simulink model "ZT_VehCtrl_18B_CAN"  (R2018b)
settings: Solver=FixedStepAuto  StartTime=0.0  StopTime=inf  FixedStep=0.005  RelTol=1e-3
InitFcn:
  | mbd_mpc_consistency_checks(bdroot(gcs));
values from neighbouring files (symbols this model uses):
  BatoverTempTh = single(80)    [VCU_INIT.m]
  BRS_PwrValid = single(5)    [VCU_INIT.m]
  BRSEnSpdTh1 = single(10)    [VCU_INIT.m]
  BRSEnSpdTh2 = single(20)    [VCU_INIT.m]
  MCUTempAlarmTh = single (60)    [VCU_INIT.m]
  mps2kmh = single(3.6)    [VCU_INIT.m]
  MtrPwrFac = single(1/9550)    [VCU_INIT.m]
  MtrTempAlarmTh = single (50)    [VCU_INIT.m]
  Padle1Signal1_Th = [PadleSignal1_min,PadleSignal1_max]    [VCU_INIT.m]
  Padle1Signal2_Th = [PadleSignal2_min,PadleSignal2_max]    [VCU_INIT.m]
  PadleSignal1_max = 3.84    [VCU_INIT.m]
  PadleSignal1_min = 0.75    [VCU_INIT.m]
  PadleSignal2_max = 1.92    [VCU_INIT.m]
  PadleSignal2_min = 0.375    [VCU_INIT.m]
  PadleValid = 0.05    [VCU_INIT.m]
  PwrLimFactor = single(0.5)    [VCU_INIT.m]
  Ratio = single(1)    [VCU_INIT.m]
  rpm2mps = single(2*pi/60 * WhlRadius/Ratio)    [VCU_INIT.m]
  SOCLowTh = single(20)    [VCU_INIT.m]
  VehPwrBackwardMax = VehPwrMax * single(0.3)    [VCU_INIT.m]
  VehPwrMax = single(MtrPwrMax * 4)    [VCU_INIT.m]
  VehTrqBackwardMax = VehTrqMax * single(0.3)    [VCU_INIT.m]
  VehTrqMax = single(MtrTrqMax * Ratio *4)    [VCU_INIT.m]
  WhlRadius = single(1)    [VCU_INIT.m]
undefined symbols (not defined in the file or in its folder): Delay_Charge, Delay_Discharge, fifo_0_vect, fifo_1_vect, LQFP, pts1_fifo_0_vect, pts1_fifo_1_vect, pts2_fifo_0_vect, pts2_fifo_1_vect, pts3_fifo_0_vect, pts3_fifo_1_vect, pts4_fifo_0_vect, pts4_fifo_1_vect
libraries: mbd_mpc574x_ec_toolbox x157, canmsglib x74, simulink x38
(part 2 of 12)

== system ZT_VehCtrl_18B_CAN/Init ==
  CAN_init : Subsystem
  Data Store Read1 : DataStoreRead  DataStoreName=VCU_Mode
  Data Store Read3 : DataStoreRead  DataStoreName=Init_flg
  If1 : If  IfExpression=u1 == 2  ShowElse=off
  If2 : If  IfExpression=u1 == 0  ShowElse=off
  Init : Subsystem
  wires:
  Data Store Read3/1 -> If2/1
  If2/1 -> Init/Action
  Data Store Read1/1 -> If1/1
  If1/1 -> CAN_init/Action

== system ZT_VehCtrl_18B_CAN/Initialization & SPI timer1 ==
  note: 由于SPI0用了两个片选，SPI3只用了一个片选（没算EEPROM）。
      | 因此直接用方波就可以了。
      | 如果增加SPI控制，建议使用StateFlow构造激活函数。
      | 由于模版使用的0.01s的仿真步长，这里构造周期为0.02s,占空比为0.5的方波。
  note: SPI3
  note: SPI0
  CS1 LS : Subsystem
  CS2 CANB : Subsystem
  CS3 LS : Subsystem
  CS5 LS : Subsystem
  Chart : Stateflow chart  TreatAsAtomicUnit=on
  Chart1 : Stateflow chart  TreatAsAtomicUnit=on
  Chart2 : Stateflow chart  TreatAsAtomicUnit=on
  Compare To Constant : simulink/Logic and Bit Operations/Compare To Constant  relop===  const=9  OutDataTypeStr=boolean
  Compare To Constant1 : simulink/Logic and Bit Operations/Compare To Constant  relop===  const=9  OutDataTypeStr=boolean
  Constant : Constant
  Data Store Read : DataStoreRead  DataStoreName=VCU_Mode
  Data Store Read1 : DataStoreRead  DataStoreName=ResetFlg
  Data Store Read2 : DataStoreRead  DataStoreName=Init_flg_SPI
  Data Store Write : DataStoreWrite  DataStoreName=VCU_Mode
  Data Store Write2 : DataStoreWrite  DataStoreName=SPI0_CS
  Data Store Write3 : DataStoreWrite  DataStoreName=SPI3_CS
  Data Store Write4 : DataStoreWrite  DataStoreName=Init_flg_SPI
  Data Type Conversion{,1..3} (4 alike) : DataTypeConversion
  If : If  IfExpression=u1 == 1  ShowElse=off
  If1 : If  IfExpression=u1 == 1  ShowElse=off
  If2 : If  IfExpression=u1 == 2  ShowElse=off
  If3 : If  IfExpression=u1 == 2  ShowElse=off
  Logical Operator : Logic  AllPortsSameDT=off  OutDataTypeStr=boolean
  Pulse Generator : DiscretePulseGenerator  PulseType=Time based  Period=0.01  PulseWidth=50
  wires:
  If/1 -> CS2 CANB/Action
  Chart/1(Flg) -> Data Type Conversion3/1
  Data Store Read2/1 -> Chart/2(InitFlg)
  If1/1 -> CS1 LS/Action
  Chart2/1(Flg) -> If3/1, [SPI3_flg], If/1
  Data Store Read/1 -> Chart2/1(VcuMode), Chart1/1(VcuMode)
  If2/1 -> CS5 LS/Action
  [SPI0_flg] -> Compare To Constant/1
  [SPI3_flg] -> Compare To Constant1/1
  Compare To Constant/1 -> Logical Operator/1
  Compare To Constant1/1 -> Logical Operator/2
  Logical Operator/1 -> Data Type Conversion2/1
  If3/1 -> CS3 LS/Action
  Pulse Generator/1 -> Data Type Conversion/1
  Constant/1 -> Data Type Conversion1/1
  Data Type Conversion/1 -> Data Store Write2/1
  Data Type Conversion1/1 -> Data Store Write3/1
  Data Type Conversion2/1 -> Data Store Write4/1
  Data Type Conversion3/1 -> Data Store Write/1
  Chart1/1(Flg) -> If1/1, [SPI0_flg], If2/1
  Data Store Read1/1 -> Chart/1(ResetFlg)

== system ZT_VehCtrl_18B_CAN/Power Managment ==
  PowerMode : Inport
  Data Type Conversion : DataTypeConversion
  HS1 : mbd_mpc574x_ec_toolbox/GPIO Blocks/Digital_Output  Priority=1  gpio_pin=PTF6: [SIUL2_GPIO86 | General Purpose IO PF[6]]  gpio_drive_strength=Disabled
  HS4 : mbd_mpc574x_ec_toolbox/GPIO Blocks/Digital_Output  Priority=1  gpio_pin=PTA13: [SIUL2_GPIO13 | General Purpose IO PA[13]]  gpio_drive_strength=Disabled
  wires:
  PowerMode/1 -> Data Type Conversion/1
  Data Type Conversion/1 -> HS4/1, HS1/1

== system ZT_VehCtrl_18B_CAN/SPI_EEPROM ==
  Data Store Memory : DataStoreMemory  DataStoreName=A_write  ReadBeforeWriteMsg=warning  WriteAfterWriteMsg=warning  WriteAfterReadMsg=warning  ShowAdditionalParam=off  OutDataTypeStr=single
      settings: RTWStateStorageClass=ExportedGlobal
  Data Store Memory10 : DataStoreMemory  DataStoreName=A_read  ReadBeforeWriteMsg=warning  WriteAfterWriteMsg=warning  WriteAfterReadMsg=warning  ShowAdditionalParam=off  OutDataTypeStr=single
      settings: RTWStateStorageClass=ExportedGlobal
  Data Store Memory18 : DataStoreMemory  DataStoreName=SPI0_CTRL0  ReadBeforeWriteMsg=warning  WriteAfterWriteMsg=warning  WriteAfterReadMsg=warning  ShowAdditionalParam=off  OutDataTypeStr=uint8
      settings: RTWStateStorageClass=ExportedGlobal
  Data Store Read : DataStoreRead  DataStoreName=SPI0_CTRL0
  SPI_read : Subsystem  TreatAsAtomicUnit=on
  SPI_write : Subsystem  TreatAsAtomicUnit=on
  Switch Case : SwitchCase  CaseConditions={1,2}  ShowDefaultCase=off
  wires:
  Data Store Read/1 -> Switch Case/1
  Switch Case/2 -> SPI_write/Action
  Switch Case/1 -> SPI_read/Action

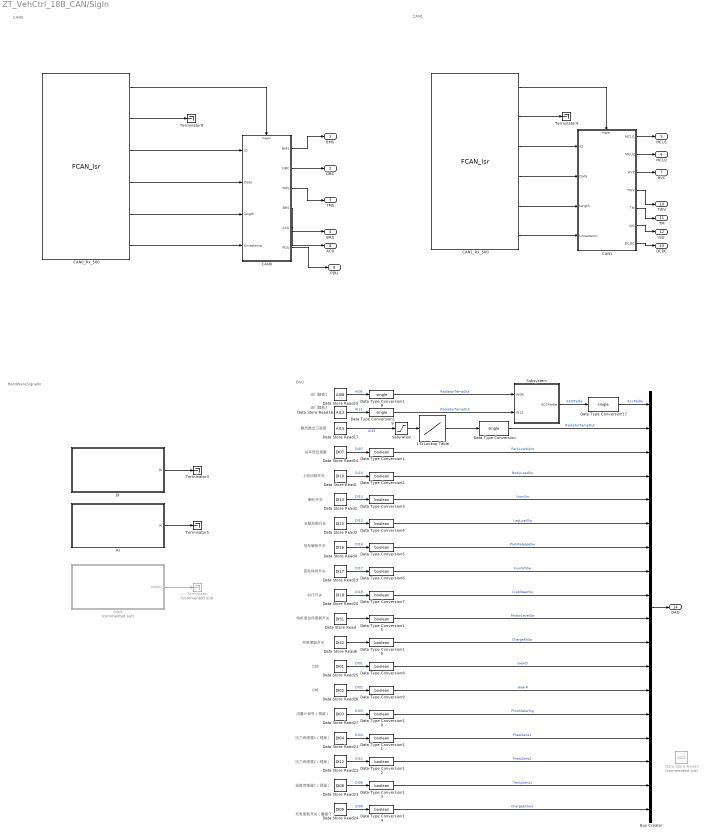
== system ZT_VehCtrl_18B_CAN/SigIn ==
  note: 充电使能开关（重复了）
  note: 温度传感器1（预留）
  note: 压力传感器2（预留）
  note: 压力传感器1（预留）
  note: 流量计信号（预留）
  note: R档
  note: D档
  note: 充电使能开关
  note: 电机液位传感器开关
  note: 斜行开关
  note: 四轮转向开关
  note: 驻车解除开关
  note: 支腿加载开关
  note: 喇叭开关
  note: 上装加载开关
  note: 驻车低压报警
  note: 散热器出口温度
  note: 油门踏板1
  note: DAQ
  note: CAN0
  note: HardWareSignalIn
  note: CAN1
  note: 油门踏板2
  1-D Lookup Table : Lookup_n-D  NumberOfTableDimensions=1  BreakpointsForDimension1=[0,5]  Table=[0,100]  InternalRulePriority=Speed  RndMeth=Simplest  InputSameDT=on
  AI : Subsystem
  Bus Creator : BusCreator  Inputs=18
  "CAN0 " : Subsystem  TreatAsAtomicUnit=on
      settings: RTWSystemCode=Nonreusable function
  CAN0_Rx_500 : mbd_mpc574x_ec_toolbox/Communication Blocks/CAN Blocks/FCAN_Isr  can_instance=0  can_event=Rx Complete
      settings: SourceProductName=NXP Model-Based Design Toolbox for MPC57xx MCUs
  CAN1 : Subsystem  TreatAsAtomicUnit=on
      settings: RTWSystemCode=Nonreusable function
  CAN1_Rx_500 : mbd_mpc574x_ec_toolbox/Communication Blocks/CAN Blocks/FCAN_Isr  can_instance=1  can_event=Rx Complete
      settings: SourceProductName=NXP Model-Based Design Toolbox for MPC57xx MCUs
  DI : Subsystem
  Data Store Read : DataStoreRead  DataStoreName=DI31
  Data Store Read1 : DataStoreRead  DataStoreName=DI10
  Data Store Read14 : DataStoreRead  DataStoreName=DI07
  Data Store Read15 : DataStoreRead  DataStoreName=AI08
  Data Store Read16 : DataStoreRead  DataStoreName=AI12
  Data Store Read17 : DataStoreRead  DataStoreName=AI15
  Data Store Read19 : DataStoreRead  DataStoreName=DI17
  Data Store Read2 : DataStoreRead  DataStoreName=DI13
  Data Store Read20 : DataStoreRead  DataStoreName=DI18
  Data Store Read21 : DataStoreRead  DataStoreName=DI04
  Data Store Read22 : DataStoreRead  DataStoreName=DI12
  Data Store Read23 : DataStoreRead  DataStoreName=DI08
  Data Store Read24 : DataStoreRead  DataStoreName=DI09
  Data Store Read25 : DataStoreRead  DataStoreName=DI01
  Data Store Read26 : DataStoreRead  DataStoreName=DI02
  Data Store Read27 : DataStoreRead  DataStoreName=DI03
  Data Store Read3 : DataStoreRead  DataStoreName=DI15
  Data Store Read4 : DataStoreRead  DataStoreName=DI16
  Data Store Read5 : DataStoreRead  Commented=on  DataStoreName=AI20
  Data Store Read6 : DataStoreRead  DataStoreName=DI32
  Data Type Conversion{,17..19} (4 alike) : DataTypeConversion  OutDataTypeStr=single
  Data Type Conversion{1..16} (16 alike) : DataTypeConversion  OutDataTypeStr=boolean
  PWM : Subsystem  Commented=on
  Saturation : Saturate
  Subsystem : Subsystem
  Terminator : Terminator  Commented=on
  Terminator{3..5,8} (4 alike) : Terminator
  BMS : Outport  VectorParamsAs1DForOutWhenUnconnected=on
  OBC : Outport  Port=2  VectorParamsAs1DForOutWhenUnconnected=on
  TMS : Outport  Port=3  VectorParamsAs1DForOutWhenUnconnected=on
  BRS : Outport  Port=4  VectorParamsAs1DForOutWhenUnconnected=on
  MCU1 : Outport  Port=5  VectorParamsAs1DForOutWhenUnconnected=on
  MCU2 : Outport  Port=6  VectorParamsAs1DForOutWhenUnconnected=on
  HVC : Outport  Port=7  VectorParamsAs1DForOutWhenUnconnected=on
  ACU : Outport  Port=8  VectorParamsAs1DForOutWhenUnconnected=on
  PDU : Outport  Port=9  VectorParamsAs1DForOutWhenUnconnected=on
  TWV : Outport  Port=10  VectorParamsAs1DForOutWhenUnconnected=on
  TM : Outport  Port=11  VectorParamsAs1DForOutWhenUnconnected=on
  ISG : Outport  Port=12  VectorParamsAs1DForOutWhenUnconnected=on
  DCDC : Outport  Port=13  VectorParamsAs1DForOutWhenUnconnected=on
  "DAQ " : Outport  Port=14
  wires:
  CAN1_Rx_500/2 -> Terminator4/1
  CAN1_Rx_500/6 -> CAN1/4(timestamp)
  CAN1_Rx_500/4 -> CAN1/2(Data)
  CAN1_Rx_500/3 -> CAN1/1(ID)
  CAN1_Rx_500/5 -> CAN1/3(length)
  CAN0_Rx_500/5 -> "CAN0 "/3(length)
  CAN0_Rx_500/3 -> "CAN0 "/1(ID)
  CAN0_Rx_500/4 -> "CAN0 "/2(Data)
  CAN0_Rx_500/6 -> "CAN0 "/4(timestamp)
  CAN0_Rx_500/1 -> "CAN0 "/Trigger
  CAN0_Rx_500/2 -> Terminator8/1
  "CAN0 "/1(BMS) -> BMS/1
  "CAN0 "/2(OBC) -> OBC/1
  "CAN0 "/4("BRS ") -> BRS/1
  "CAN0 "/3(TMS) -> TMS/1
  CAN1_Rx_500/1 -> CAN1/Trigger
  PWM/1(PWMIn) -> Terminator/1
  DI/1(DI) -> Terminator3/1
  AI/1(AI) -> Terminator5/1
  CAN1/1(MCU1) -> MCU1/1
  CAN1/3(HVC) -> HVC/1
  CAN1/5(TM) -> TM/1
  CAN1/6("ISG ") -> ISG/1
  CAN1/4(TWV) -> TWV/1
  "CAN0 "/6(PDU) -> PDU/1
  "CAN0 "/5(ACU) -> ACU/1
  CAN1/2(MCU2) -> MCU2/1
  CAN1/7(DCDC) -> DCDC/1
  Data Store Read15/1 -> Data Type Conversion18/1  "AI08"
  Data Store Read16/1 -> Data Type Conversion19/1  "AI12"
  Subsystem/1("ACCPadle ") -> Data Type Conversion17/1  "ACCPadle"
  Saturation/1 -> 1-D Lookup Table/1
  Data Store Read17/1 -> Saturation/1  "AI15"
  1-D Lookup Table/1 -> Data Type Conversion/1
  Data Type Conversion/1 -> Bus Creator/2  "RadiatorTempOut"
  Data Store Read14/1 -> Data Type Conversion1/1  "DI07"
  Data Store Read1/1 -> Data Type Conversion2/1  "DI10"
  Data Store Read2/1 -> Data Type Conversion3/1  "DI13"
  Data Store Read3/1 -> Data Type Conversion4/1  "DI15"
  Data Store Read4/1 -> Data Type Conversion5/1  "DI16"
  Data Store Read19/1 -> Data Type Conversion6/1  "DI17"
  Data Store Read20/1 -> Data Type Conversion7/1  "DI18"
  Data Store Read25/1 -> Data Type Conversion8/1  "DI01"
  Data Store Read26/1 -> Data Type Conversion9/1  "DI02"
  Data Store Read27/1 -> Data Type Conversion10/1  "DI03"
  Data Store Read24/1 -> Data Type Conversion14/1  "DI09"
  Data Store Read23/1 -> Data Type Conversion13/1  "DI08"
  Data Store Read22/1 -> Data Type Conversion12/1  "DI12"
  Data Store Read21/1 -> Data Type Conversion11/1  "DI04"
  Data Type Conversion1/1 -> Bus Creator/3  "ParkLowWarn"
  Data Type Conversion2/1 -> Bus Creator/4  "BodyLoadSw"
  Data Type Conversion3/1 -> Bus Creator/5  "HornSw"
  Data Type Conversion4/1 -> Bus Creator/6  "LegLoadSw"
  Data Type Conversion5/1 -> Bus Creator/7  "ParkReleaseSw"
  Data Type Conversion6/1 -> Bus Creator/8  "FourWSSw"
  Data Type Conversion7/1 -> Bus Creator/9  "CrabSteerSw"
  Data Type Conversion8/1 -> Bus Creator/12  "GearD"
  Data Type Conversion9/1 -> Bus Creator/13  "GearR"
  Data Type Conversion10/1 -> Bus Creator/14  "FlowMeterSig"
  Data Type Conversion11/1 -> Bus Creator/15  "PressSens1"
  Data Type Conversion12/1 -> Bus Creator/16  "PressSens2"
  Data Type Conversion13/1 -> Bus Creator/17  "TempSens1"
  Data Type Conversion14/1 -> Bus Creator/18  "ChargeEnSw2"
  Bus Creator/1 -> "DAQ "/1
  Data Store Read/1 -> Data Type Conversion15/1
  Data Store Read6/1 -> Data Type Conversion16/1
  Data Type Conversion15/1 -> Bus Creator/10  "MotorLevelSw"
  Data Type Conversion16/1 -> Bus Creator/11  "ChargeEnSw"
  Data Type Conversion17/1 -> Bus Creator/1  "AccPadle"
  Data Type Conversion18/1 -> Subsystem/1(AI08)  "RadiatorTempOut"
  Data Type Conversion19/1 -> Subsystem/2(AI12)  "RadiatorTempOut"

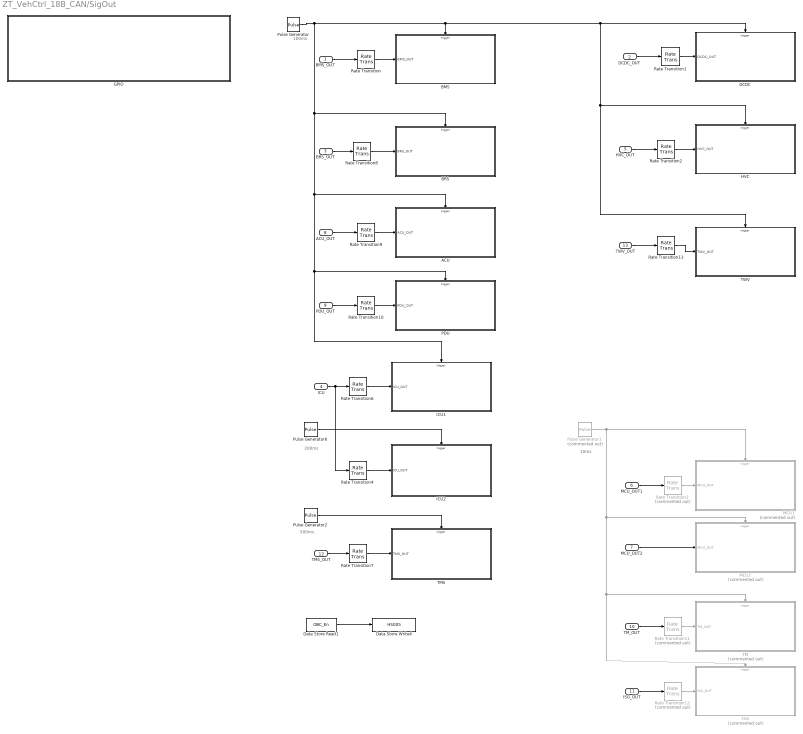
== system ZT_VehCtrl_18B_CAN/SigOut ==
  note: 10ms
  note: 500ms
  note: 100ms
  note: 200ms
  BMS_OUT : Inport
  "DCDC_OUT " : Inport  Port=2
  BRS_OUT : Inport  Port=3
  ICU : Inport  Port=4
  HVC_OUT : Inport  Port=5
  MCU_OUT1 : Inport  Port=6
  MCU_OUT2 : Inport  Port=7
  ACU_OUT : Inport  Port=8
  PDU_OUT : Inport  Port=9
  TM_OUT : Inport  Port=10
  ISG_OUT : Inport  Port=11
  TMS_OUT : Inport  Port=12
  TWV_OUT : Inport  Port=13
  ACU : Subsystem  TreatAsAtomicUnit=on  SystemSampleTime=0.01
  BMS : Subsystem  TreatAsAtomicUnit=on  SystemSampleTime=0.01
  BRS : Subsystem  TreatAsAtomicUnit=on  SystemSampleTime=0.01
  DCDC : Subsystem  TreatAsAtomicUnit=on  SystemSampleTime=0.01
  Data Store Read1 : DataStoreRead  DataStoreName=OBC_En
  Data Store Write4 : DataStoreWrite  DataStoreName=HS005
  "GPIO " : Subsystem
  HVC : Subsystem  TreatAsAtomicUnit=on  SystemSampleTime=0.01
  "ICU1 " : Subsystem  TreatAsAtomicUnit=on  SystemSampleTime=0.01
  ICU2 : Subsystem  TreatAsAtomicUnit=on  SystemSampleTime=0.01
  ISG : Subsystem  Commented=on  TreatAsAtomicUnit=on  SystemSampleTime=0.01
  MCU1 : Subsystem  Commented=on  TreatAsAtomicUnit=on  SystemSampleTime=0.01
  MCU2 : Subsystem  Commented=on  TreatAsAtomicUnit=on  SystemSampleTime=0.01
  PDU : Subsystem  TreatAsAtomicUnit=on  SystemSampleTime=0.01
  Pulse Generator : DiscretePulseGenerator  PulseType=Time based  Period=0.1  PulseWidth=50
  Pulse Generator1 : DiscretePulseGenerator  Commented=on  PulseType=Time based  Period=0.01  PulseWidth=50
  Pulse Generator2 : DiscretePulseGenerator  PulseType=Time based  Period=0.5  PulseWidth=50
  Pulse Generator6 : DiscretePulseGenerator  PulseType=Time based  Period=0.2  PulseWidth=50
  Rate Transition{,1..2,4,6..10,13} (10 alike) : RateTransition
  Rate Transition11 : RateTransition  Commented=on
  Rate Transition12 : RateTransition  Commented=on
  Rate Transition3 : RateTransition  Commented=on
  TM : Subsystem  Commented=on  TreatAsAtomicUnit=on  SystemSampleTime=0.01
  TMS : Subsystem  TreatAsAtomicUnit=on  SystemSampleTime=0.01
  TWV : Subsystem  TreatAsAtomicUnit=on  SystemSampleTime=0.01
  wires:
  BMS_OUT/1 -> Rate Transition/1
  Rate Transition/1 -> BMS/1("BMS_OUT ")
  Rate Transition4/1 -> ICU2/1("ICU_OUT ")
  Pulse Generator/1 -> "ICU1 "/Trigger, PDU/Trigger, ACU/Trigger, BRS/Trigger, DCDC/Trigger, HVC/Trigger, TWV/Trigger, BMS/Trigger
  ICU/1 -> Rate Transition4/1, Rate Transition6/1
  Rate Transition6/1 -> "ICU1 "/1("ICU_OUT ")
  TMS_OUT/1 -> Rate Transition7/1
  Rate Transition7/1 -> TMS/1("TMS_OUT ")
  BRS_OUT/1 -> Rate Transition8/1
  Rate Transition8/1 -> BRS/1("BRS_OUT ")
  Rate Transition1/1 -> DCDC/1("DCDC_OUT ")
  "DCDC_OUT "/1 -> Rate Transition1/1
  HVC_OUT/1 -> Rate Transition2/1
  Rate Transition2/1 -> HVC/1("HVC_OUT ")
  Rate Transition3/1 -> MCU1/1("MCU_OUT ")
  MCU_OUT1/1 -> Rate Transition3/1
  Rate Transition9/1 -> ACU/1("ACU_OUT ")
  ACU_OUT/1 -> Rate Transition9/1
  PDU_OUT/1 -> Rate Transition10/1
  Rate Transition10/1 -> PDU/1("PDU_OUT ")
  TM_OUT/1 -> Rate Transition11/1
  Rate Transition11/1 -> TM/1("TM_OUT ")
  Rate Transition12/1 -> ISG/1("ISG_OUT ")
  ISG_OUT/1 -> Rate Transition12/1
  Pulse Generator1/1 -> MCU2/Trigger, ISG/Trigger, TM/Trigger, MCU1/Trigger
  Rate Transition13/1 -> TWV/1("TWV_OUT ")
  TWV_OUT/1 -> Rate Transition13/1
  Pulse Generator2/1 -> TMS/Trigger
  Pulse Generator6/1 -> ICU2/Trigger
  MCU_OUT2/1 -> MCU2/1("MCU_OUT ")
  Data Store Read1/1 -> Data Store Write4/1

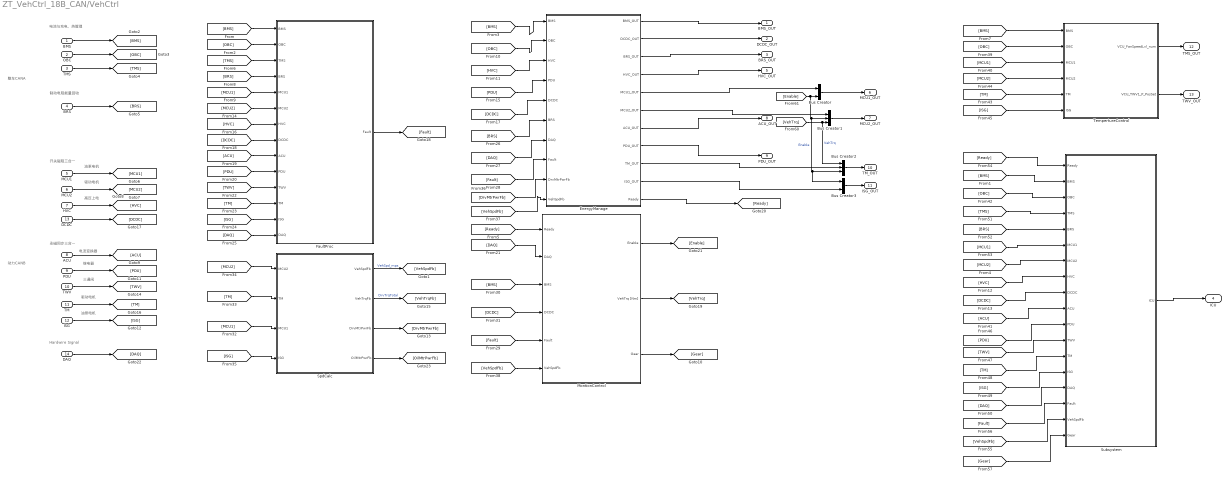
== system ZT_VehCtrl_18B_CAN/VehCtrl ==
  note: 动力CANB
  note: 整车CANA
  note: Hardwire Signal
  note: 油泵电机
  note: 驱动电机
  note: 三通阀
  note: 继电器
  note: 电流变换器
  note: 永磁同步三合一
  note: 高压上电
  note: 驱动电机
  note: 油泵电机
  note: 开关磁阻三合一
  note: 制动电阻能量回收
  note: 电池与充电、热管理
  "BMS " : Inport
  "OBC " : Inport  Port=2
  "TMS " : Inport  Port=3
  BRS : Inport  Port=4
  "MCU1 " : Inport  Port=5
  "MCU2 " : Inport  Port=6
  "HVC " : Inport  Port=7
  ACU : Inport  Port=8
  PDU : Inport  Port=9
  "TWV " : Inport  Port=10
  TM : Inport  Port=11
  "ISG " : Inport  Port=12
  "DCDC " : Inport  Port=13
  "DAQ " : Inport  Port=14
  Bus Creator : BusCreator  Inputs=2
  Bus Creator1 : BusCreator  Inputs=3
  Bus Creator2 : BusCreator  Inputs=3
  Bus Creator3 : BusCreator  Inputs=2
  EnergyManage : Subsystem
  FaultProc : Subsystem
  MontionControl : Subsystem
  SpdCalc : Subsystem
  Subsystem : Subsystem
  TempertureControl : Subsystem
  BMS_OUT : Outport
  DCDC_OUT : Outport  Port=2
  BRS_OUT : Outport  Port=3
  ICU : Outport  Port=4
  HVC_OUT : Outport  Port=5
  MCU1_OUT : Outport  Port=6
  MCU2_OUT : Outport  Port=7
  ACU_OUT : Outport  Port=8
  PDU_OUT : Outport  Port=9
  TM_OUT : Outport  Port=10
  ISG_OUT : Outport  Port=11
  "TMS_OUT " : Outport  Port=12
  TWV_OUT : Outport  Port=13
  wires:
  [OBC] -> FaultProc/2("OBC ")
  [TMS] -> FaultProc/3("TMS ")
  [BRS] -> FaultProc/4("BRS ")
  [MCU1] -> FaultProc/5("MCU1 ")
  FaultProc/1("Fault ") -> [Fault]
  EnergyManage/1("BMS_OUT ") -> BMS_OUT/1
  EnergyManage/2("DCDC_OUT ") -> DCDC_OUT/1
  [BMS] -> FaultProc/1("BMS ")
  SpdCalc/2("VehTrqFb ") -> [VehTrqFb]  "DrvTrqTotal"
  SpdCalc/4("OilMtrPwrFb ") -> [OilMtrPwrFb]
  SpdCalc/3("DrvMtrPwrFb ") -> [DrvMtrPwrFb]
  SpdCalc/1(VehSpdFb) -> [VehSpdFb]  "VehSpd_mps"
  Subsystem/1(ICU) -> ICU/1
  "BMS "/1 -> [BMS]
  "OBC "/1 -> [OBC]
  "TMS "/1 -> [TMS]
  BRS/1 -> [BRS]
  "MCU1 "/1 -> [MCU1]
  "MCU2 "/1 -> [MCU2]
  "HVC "/1 -> [HVC]
  ACU/1 -> [ACU]
  PDU/1 -> [PDU]
  "TWV "/1 -> [TWV]
  TM/1 -> [TM]
  "ISG "/1 -> [ISG]
  "DCDC "/1 -> [DCDC]
  "DAQ "/1 -> [DAQ]
  [MCU2] -> FaultProc/6(MCU2)
  [HVC] -> FaultProc/7(HVC)
  [DCDC] -> FaultProc/8(DCDC)
  [ACU] -> FaultProc/9(ACU)
  [PDU] -> FaultProc/10(PDU)
  [TWV] -> FaultProc/11(TWV)
  [TM] -> FaultProc/12(TM)
  [ISG] -> FaultProc/13(ISG)
  [DAQ] -> FaultProc/14(DAQ)
  [BMS] -> EnergyManage/1(BMS)
  [OBC] -> EnergyManage/2(OBC)
  [HVC] -> EnergyManage/3(HVC)
  [PDU] -> EnergyManage/4(PDU)
  [DCDC] -> EnergyManage/5(DCDC)
  [BRS] -> EnergyManage/6(BRS)
  [DAQ] -> EnergyManage/7(DAQ)
  [Fault] -> EnergyManage/8(Fault)
  EnergyManage/3(BRS_OUT) -> BRS_OUT/1
  EnergyManage/4(HVC_OUT) -> HVC_OUT/1
  EnergyManage/7(ACU_OUT) -> ACU_OUT/1
  EnergyManage/8(PDU_OUT) -> PDU_OUT/1
  EnergyManage/11(Ready) -> [Ready]
  [Ready] -> MontionControl/1(Ready)
  [DAQ] -> MontionControl/2(DAQ)
  [Fault] -> MontionControl/5(Fault)
  [BMS] -> MontionControl/3(BMS)
  [DCDC] -> MontionControl/4(DCDC)
  [TM] -> SpdCalc/2(TM)
  [ISG] -> SpdCalc/4(ISG)
  [MCU1] -> SpdCalc/3(MCU1)
  [MCU2] -> SpdCalc/1(MCU2)
  [DrvMtrPwrFb] -> EnergyManage/9(DrvMtrPwrFb)
  [VehSpdFb] -> EnergyManage/10(VehSpdFb)
  [VehSpdFb] -> MontionControl/6(VehSpdFb)
  [BMS] -> TempertureControl/1(BMS)
  [OBC] -> TempertureControl/2(OBC)
  [MCU1] -> TempertureControl/3(MCU1)
  [MCU2] -> TempertureControl/4(MCU2)
  [TM] -> TempertureControl/5(TM)
  [ISG] -> TempertureControl/6(ISG)
  TempertureControl/1(VCU_FanSpeedLvl_num) -> "TMS_OUT "/1
  TempertureControl/2(VCU_TWV1_P_PosSet) -> TWV_OUT/1
  [Ready] -> Subsystem/1(Ready)
  [BMS] -> Subsystem/2(BMS)
  [OBC] -> Subsystem/3(OBC)
  [TMS] -> Subsystem/4(TMS)
  [BRS] -> Subsystem/5(BRS)
  [MCU1] -> Subsystem/6(MCU1)
  [MCU2] -> Subsystem/7(MCU2)
  [HVC] -> Subsystem/8(HVC)
  [DCDC] -> Subsystem/9(DCDC)
  [ACU] -> Subsystem/10(ACU)
  [PDU] -> Subsystem/11(PDU)
  [TWV] -> Subsystem/12(TWV)
  [TM] -> Subsystem/13(TM)
  [ISG] -> Subsystem/14(ISG)
  [DAQ] -> Subsystem/15(DAQ)
  [Fault] -> Subsystem/16(Fault)
  [VehSpdFb] -> Subsystem/17(VehSpdFb)
  MontionControl/3(Gear) -> [Gear]
  [Gear] -> Subsystem/18(Gear)
  MontionControl/2(VehTrq [Nm]) -> [VehTrq]
  MontionControl/1(Enable) -> [Enable]
  Bus Creator/1 -> MCU1_OUT/1
  EnergyManage/5(MCU1_OUT) -> Bus Creator/1
  [Enable] -> Bus Creator3/1, Bus Creator2/3, Bus Creator1/2, Bus Creator/2  "Enable"
  EnergyManage/6(MCU2_OUT) -> Bus Creator1/1
  [VehTrq] -> Bus Creator2/1, Bus Creator1/3  "VehTrq"
  Bus Creator1/1 -> MCU2_OUT/1
  Bus Creator2/1 -> TM_OUT/1
  EnergyManage/9(TM_OUT) -> Bus Creator2/2
  Bus Creator3/1 -> ISG_OUT/1
  EnergyManage/10(ISG_OUT) -> Bus Creator3/2

== system ZT_VehCtrl_18B_CAN/Init/CAN_init ==
  note: CAN2
  note: CAN1
  Action Port : ActionPort  ActionType=then
  ACU1 : mbd_mpc574x_ec_toolbox/Communication Blocks/CAN Blocks/FCAN_Receive  can_instance=0  can_mode=Non-blocking  can_timeout_ms=0  can_mb_idx=36  can_extended_id=on  can_is_remote=off  can_id=0C08A79A  can_msg_mask=FFFFFFFF  show_adv_opts=off  can_use_rxfifo=off  can_fd_enable=off
      settings: SourceProductName=NXP Model-Based Design Toolbox for MPC57xx MCUs
  ACU2 : mbd_mpc574x_ec_toolbox/Communication Blocks/CAN Blocks/FCAN_Receive  can_instance=0  can_mode=Non-blocking  can_timeout_ms=0  can_mb_idx=37  can_extended_id=on  can_is_remote=off  can_id=0C09A79B  can_msg_mask=FFFFFFFF  show_adv_opts=off  can_use_rxfifo=off  can_fd_enable=off
      settings: SourceProductName=NXP Model-Based Design Toolbox for MPC57xx MCUs
  ACU3 : mbd_mpc574x_ec_toolbox/Communication Blocks/CAN Blocks/FCAN_Receive  can_instance=0  can_mode=Non-blocking  can_timeout_ms=0  can_mb_idx=38  can_extended_id=on  can_is_remote=off  can_id=0C0AA79D  can_msg_mask=FFFFFFFF  show_adv_opts=off  can_use_rxfifo=off  can_fd_enable=off
      settings: SourceProductName=NXP Model-Based Design Toolbox for MPC57xx MCUs
  BMS Power Infor : mbd_mpc574x_ec_toolbox/Communication Blocks/CAN Blocks/FCAN_Receive  can_instance=0  can_mode=Non-blocking  can_timeout_ms=0  can_mb_idx=3  can_extended_id=off  can_is_remote=off  can_id=211  can_msg_mask=FFFFFFFF  show_adv_opts=off  can_use_rxfifo=off  can_fd_enable=off
      settings: SourceProductName=NXP Model-Based Design Toolbox for MPC57xx MCUs
  BMS Statistic_Temperature of Battery : mbd_mpc574x_ec_toolbox/Communication Blocks/CAN Blocks/FCAN_Receive  can_instance=0  can_mode=Non-blocking  can_timeout_ms=0  can_mb_idx=5  can_extended_id=off  can_is_remote=off  can_id=353  can_msg_mask=FFFFFFFF  show_adv_opts=off  can_use_rxfifo=off  can_fd_enable=off
      settings: SourceProductName=NXP Model-Based Design Toolbox for MPC57xx MCUs
  BMS other Information3 : mbd_mpc574x_ec_toolbox/Communication Blocks/CAN Blocks/FCAN_Receive  can_instance=0  can_mode=Non-blocking  can_timeout_ms=0  can_mb_idx=6  can_extended_id=off  can_is_remote=off  can_id=205  can_msg_mask=FFFFFFFF  show_adv_opts=off  can_use_rxfifo=off  can_fd_enable=off
      settings: SourceProductName=NXP Model-Based Design Toolbox for MPC57xx MCUs
  BMSWarning Status : mbd_mpc574x_ec_toolbox/Communication Blocks/CAN Blocks/FCAN_Receive  can_instance=0  can_mode=Non-blocking  can_timeout_ms=0  can_mb_idx=2  can_extended_id=off  can_is_remote=off  can_id=1F5  can_msg_mask=FFFFFFFF  show_adv_opts=off  can_use_rxfifo=off  can_fd_enable=off
      settings: SourceProductName=NXP Model-Based Design Toolbox for MPC57xx MCUs
  BMS_Information 1 : mbd_mpc574x_ec_toolbox/Communication Blocks/CAN Blocks/FCAN_Receive  can_instance=0  can_mode=Non-blocking  can_timeout_ms=0  can_mb_idx=0  can_extended_id=off  can_is_remote=off  can_id=1E1  can_msg_mask=FFFFFFFF  show_adv_opts=off  can_use_rxfifo=off  can_fd_enable=off
      settings: SourceProductName=NXP Model-Based Design Toolbox for MPC57xx MCUs
  BMS_Information 2 : mbd_mpc574x_ec_toolbox/Communication Blocks/CAN Blocks/FCAN_Receive  can_instance=0  can_mode=Non-blocking  can_timeout_ms=0  can_mb_idx=1  can_extended_id=off  can_is_remote=off  can_id=1E4  can_msg_mask=FFFFFFFF  show_adv_opts=off  can_use_rxfifo=off  can_fd_enable=off
      settings: SourceProductName=NXP Model-Based Design Toolbox for MPC57xx MCUs
  BRS2VCU1 : mbd_mpc574x_ec_toolbox/Communication Blocks/CAN Blocks/FCAN_Receive  can_instance=0  can_mode=Non-blocking  can_timeout_ms=0  can_mb_idx=11  can_extended_id=on  can_is_remote=off  can_id=18FE25E4  can_msg_mask=FFFFFFFF  show_adv_opts=off  can_use_rxfifo=off  can_fd_enable=off
      settings: SourceProductName=NXP Model-Based Design Toolbox for MPC57xx MCUs
  BRS2VCU2 : mbd_mpc574x_ec_toolbox/Communication Blocks/CAN Blocks/FCAN_Receive  can_instance=0  can_mode=Non-blocking  can_timeout_ms=0  can_mb_idx=12  can_extended_id=on  can_is_remote=off  can_id=18FE26E4  can_msg_mask=FFFFFFFF  show_adv_opts=off  can_use_rxfifo=off  can_fd_enable=off
      settings: SourceProductName=NXP Model-Based Design Toolbox for MPC57xx MCUs
  BRS2VCU3 : mbd_mpc574x_ec_toolbox/Communication Blocks/CAN Blocks/FCAN_Receive  can_instance=0  can_mode=Non-blocking  can_timeout_ms=0  can_mb_idx=13  can_extended_id=on  can_is_remote=off  can_id=18FE27E4  can_msg_mask=FFFFFFFF  show_adv_opts=off  can_use_rxfifo=off  can_fd_enable=off
      settings: SourceProductName=NXP Model-Based Design Toolbox for MPC57xx MCUs
  DCDC1_1 : mbd_mpc574x_ec_toolbox/Communication Blocks/CAN Blocks/FCAN_Receive  can_instance=1  can_mode=Non-blocking  can_timeout_ms=0  can_mb_idx=24  can_extended_id=on  can_is_remote=off  can_id=1800D08F  can_msg_mask=FFFFFFFF  show_adv_opts=off  can_use_rxfifo=off  can_fd_enable=off
      settings: SourceProductName=NXP Model-Based Design Toolbox for MPC57xx MCUs
  DCDC1_2 : mbd_mpc574x_ec_toolbox/Communication Blocks/CAN Blocks/FCAN_Receive  can_instance=1  can_mode=Non-blocking  can_timeout_ms=0  can_mb_idx=26  can_extended_id=on  can_is_remote=off  can_id=1801D08F  can_msg_mask=FFFFFFFF  show_adv_opts=off  can_use_rxfifo=off  can_fd_enable=off
      settings: SourceProductName=NXP Model-Based Design Toolbox for MPC57xx MCUs
  HVC1_LV : mbd_mpc574x_ec_toolbox/Communication Blocks/CAN Blocks/FCAN_Receive  can_instance=1  can_mode=Non-blocking  can_timeout_ms=0  can_mb_idx=25  can_extended_id=on  can_is_remote=off  can_id=180105A1  can_msg_mask=FFFFFFFF  show_adv_opts=off  can_use_rxfifo=off  can_fd_enable=off
      settings: SourceProductName=NXP Model-Based Design Toolbox for MPC57xx MCUs
  HVC3_Temp : mbd_mpc574x_ec_toolbox/Communication Blocks/CAN Blocks/FCAN_Receive  can_instance=1  can_mode=Non-blocking  can_timeout_ms=0  can_mb_idx=27  can_extended_id=on  can_is_remote=off  can_id=180305A1  can_msg_mask=FFFFFFFF  show_adv_opts=off  can_use_rxfifo=off  can_fd_enable=off
      settings: SourceProductName=NXP Model-Based Design Toolbox for MPC57xx MCUs
  HVC4_RlySt : mbd_mpc574x_ec_toolbox/Communication Blocks/CAN Blocks/FCAN_Receive  can_instance=1  can_mode=Non-blocking  can_timeout_ms=0  can_mb_idx=28  can_extended_id=on  can_is_remote=off  can_id=180405A1  can_msg_mask=FFFFFFFF  show_adv_opts=off  can_use_rxfifo=off  can_fd_enable=off
      settings: SourceProductName=NXP Model-Based Design Toolbox for MPC57xx MCUs
  HVC7_HV1 : mbd_mpc574x_ec_toolbox/Communication Blocks/CAN Blocks/FCAN_Receive  can_instance=1  can_mode=Non-blocking  can_timeout_ms=0  can_mb_idx=29  can_extended_id=on  can_is_remote=off  can_id=180705A1  can_msg_mask=FFFFFFFF  show_adv_opts=off  can_use_rxfifo=off  can_fd_enable=off
      settings: SourceProductName=NXP Model-Based Design Toolbox for MPC57xx MCUs
  ISG MCU STATUS1 : mbd_mpc574x_ec_toolbox/Communication Blocks/CAN Blocks/FCAN_Receive  can_instance=1  can_mode=Non-blocking  can_timeout_ms=0  can_mb_idx=43  can_extended_id=on  can_is_remote=off  can_id=CFF0006  can_msg_mask=FFFFFFFF  show_adv_opts=off  can_use_rxfifo=off  can_fd_enable=off
      settings: SourceProductName=NXP Model-Based Design Toolbox for MPC57xx MCUs
  ISG MCU STATUS2 : mbd_mpc574x_ec_toolbox/Communication Blocks/CAN Blocks/FCAN_Receive  can_instance=1  can_mode=Non-blocking  can_timeout_ms=0  can_mb_idx=44  can_extended_id=on  can_is_remote=off  can_id=CFF0106  can_msg_mask=FFFFFFFF  show_adv_opts=off  can_use_rxfifo=off  can_fd_enable=off
      settings: SourceProductName=NXP Model-Based Design Toolbox for MPC57xx MCUs
  ISG MCU STATUS3 : mbd_mpc574x_ec_toolbox/Communication Blocks/CAN Blocks/FCAN_Receive  can_instance=1  can_mode=Non-blocking  can_timeout_ms=0  can_mb_idx=45  can_extended_id=on  can_is_remote=off  can_id=CFF0206  can_msg_mask=FFFFFFFF  show_adv_opts=off  can_use_rxfifo=off  can_fd_enable=off
      settings: SourceProductName=NXP Model-Based Design Toolbox for MPC57xx MCUs
  MCU1Msg1 : mbd_mpc574x_ec_toolbox/Communication Blocks/CAN Blocks/FCAN_Receive  can_instance=1  can_mode=Non-blocking  can_timeout_ms=0  can_mb_idx=30  can_extended_id=on  can_is_remote=off  can_id=1836D0EF  can_msg_mask=FFFFFFFF  show_adv_opts=off  can_use_rxfifo=off  can_fd_enable=off
      settings: SourceProductName=NXP Model-Based Design Toolbox for MPC57xx MCUs
  MCU1Msg2 : mbd_mpc574x_ec_toolbox/Communication Blocks/CAN Blocks/FCAN_Receive  can_instance=1  can_mode=Non-blocking  can_timeout_ms=0  can_mb_idx=31  can_extended_id=on  can_is_remote=off  can_id=1837D0EF  can_msg_mask=FFFFFFFF  show_adv_opts=off  can_use_rxfifo=off  can_fd_enable=off
      settings: SourceProductName=NXP Model-Based Design Toolbox for MPC57xx MCUs
  MCU1Msg3 : mbd_mpc574x_ec_toolbox/Communication Blocks/CAN Blocks/FCAN_Receive  can_instance=1  can_mode=Non-blocking  can_timeout_ms=0  can_mb_idx=32  can_extended_id=on  can_is_remote=off  can_id=1838D0EF  can_msg_mask=FFFFFFFF  show_adv_opts=off  can_use_rxfifo=off  can_fd_enable=off
      settings: SourceProductName=NXP Model-Based Design Toolbox for MPC57xx MCUs
  MCU2Msg1 : mbd_mpc574x_ec_toolbox/Communication Blocks/CAN Blocks/FCAN_Receive  can_instance=1  can_mode=Non-blocking  can_timeout_ms=0  can_mb_idx=33  can_extended_id=on  can_is_remote=off  can_id=1836D0F1  can_msg_mask=FFFFFFFF  show_adv_opts=off  can_use_rxfifo=off  can_fd_enable=off
      settings: SourceProductName=NXP Model-Based Design Toolbox for MPC57xx MCUs
  MCU2Msg2 : mbd_mpc574x_ec_toolbox/Communication Blocks/CAN Blocks/FCAN_Receive  can_instance=1  can_mode=Non-blocking  can_timeout_ms=0  can_mb_idx=34  can_extended_id=on  can_is_remote=off  can_id=1837D0F1  can_msg_mask=FFFFFFFF  show_adv_opts=off  can_use_rxfifo=off  can_fd_enable=off
      settings: SourceProductName=NXP Model-Based Design Toolbox for MPC57xx MCUs
  MCU2Msg3 : mbd_mpc574x_ec_toolbox/Communication Blocks/CAN Blocks/FCAN_Receive  can_instance=1  can_mode=Non-blocking  can_timeout_ms=0  can_mb_idx=35  can_extended_id=on  can_is_remote=off  can_id=1838D0F1  can_msg_mask=FFFFFFFF  show_adv_opts=off  can_use_rxfifo=off  can_fd_enable=off
      settings: SourceProductName=NXP Model-Based Design Toolbox for MPC57xx MCUs
  OBC_Charger Status : mbd_mpc574x_ec_toolbox/Communication Blocks/CAN Blocks/FCAN_Receive  can_instance=0  can_mode=Non-blocking  can_timeout_ms=0  can_mb_idx=9  can_extended_id=off  can_is_remote=off  can_id=220  can_msg_mask=FFFFFFFF  show_adv_opts=off  can_use_rxfifo=off  can_fd_enable=off
      settings: SourceProductName=NXP Model-Based Design Toolbox for MPC57xx MCUs
  PDU_RelaySts : mbd_mpc574x_ec_toolbox/Communication Blocks/CAN Blocks/FCAN_Receive  can_instance=0  can_mode=Non-blocking  can_timeout_ms=0  can_mb_idx=39  can_extended_id=on  can_is_remote=off  can_id=18FF2BC8  can_msg_mask=FFFFFFFF  show_adv_opts=off  can_use_rxfifo=off  can_fd_enable=off
      settings: SourceProductName=NXP Model-Based Design Toolbox for MPC57xx MCUs
  TM MCU STATUS1 : mbd_mpc574x_ec_toolbox/Communication Blocks/CAN Blocks/FCAN_Receive  can_instance=1  can_mode=Non-blocking  can_timeout_ms=0  can_mb_idx=40  can_extended_id=on  can_is_remote=off  can_id=CFF0005  can_msg_mask=FFFFFFFF  show_adv_opts=off  can_use_rxfifo=off  can_fd_enable=off
      settings: SourceProductName=NXP Model-Based Design Toolbox for MPC57xx MCUs
  TM MCU STATUS2 : mbd_mpc574x_ec_toolbox/Communication Blocks/CAN Blocks/FCAN_Receive  can_instance=1  can_mode=Non-blocking  can_timeout_ms=0  can_mb_idx=41  can_extended_id=on  can_is_remote=off  can_id=CFF0105  can_msg_mask=FFFFFFFF  show_adv_opts=off  can_use_rxfifo=off  can_fd_enable=off
      settings: SourceProductName=NXP Model-Based Design Toolbox for MPC57xx MCUs
  TM MCU STATUS3 : mbd_mpc574x_ec_toolbox/Communication Blocks/CAN Blocks/FCAN_Receive  can_instance=1  can_mode=Non-blocking  can_timeout_ms=0  can_mb_idx=42  can_extended_id=on  can_is_remote=off  can_id=CFF0205  can_msg_mask=FFFFFFFF  show_adv_opts=off  can_use_rxfifo=off  can_fd_enable=off
      settings: SourceProductName=NXP Model-Based Design Toolbox for MPC57xx MCUs
  TMS2VCU : mbd_mpc574x_ec_toolbox/Communication Blocks/CAN Blocks/FCAN_Receive  can_instance=0  can_mode=Non-blocking  can_timeout_ms=0  can_mb_idx=10  can_extended_id=on  can_is_remote=off  can_id=18FFF346  can_msg_mask=FFFFFFFF  show_adv_opts=off  can_use_rxfifo=off  can_fd_enable=off
      settings: SourceProductName=NXP Model-Based Design Toolbox for MPC57xx MCUs
  TWV : mbd_mpc574x_ec_toolbox/Communication Blocks/CAN Blocks/FCAN_Receive  can_instance=1  can_mode=Non-blocking  can_timeout_ms=0  can_mb_idx=46  can_extended_id=on  can_is_remote=off  can_id=18FF243B  can_msg_mask=FFFFFFFF  show_adv_opts=off  can_use_rxfifo=off  can_fd_enable=off
      settings: SourceProductName=NXP Model-Based Design Toolbox for MPC57xx MCUs

== system ZT_VehCtrl_18B_CAN/Init/Init ==
  note: MainRelay
  Action Port : ActionPort  ActionType=then
  Constant : Constant
  Constant2 : Constant
  Data Store Write : DataStoreWrite  DataStoreName=LS001
  Data Store Write3 : DataStoreWrite  DataStoreName=Init_flg
  Data Type Conversion : DataTypeConversion
  Data Type Conversion2 : DataTypeConversion
  wires:
  Constant/1 -> Data Type Conversion/1
  Data Type Conversion/1 -> Data Store Write3/1
  Constant2/1 -> Data Type Conversion2/1
  Data Type Conversion2/1 -> Data Store Write/1

== system ZT_VehCtrl_18B_CAN/Initialization & SPI timer1/CS1 LS ==
  Action Port : ActionPort  ActionType=then
  Chart : Stateflow chart  TreatAsAtomicUnit=on
  Data Type Conversion{,1,3..4} (4 alike) : DataTypeConversion
  Demux1 : Demux  Outputs=2
  SPI_Master_Transfer_To1 : mbd_mpc574x_ec_toolbox/Communication Blocks/SPI Blocks/SPI_Master_Transfer  Priority=2  InstanceNumber=0  xfermode=Non blocking  timeout=50  spi_upd=on  WhichPCS=5
  Subsystem : Subsystem  Commented=on
  Terminator : Terminator
  Terminator1 : Terminator
  Vector Concatenate1 : Concatenate
  wires:
  SPI_Master_Transfer_To1/1 -> Demux1/1
  Data Type Conversion3/1 -> Terminator/1
  Vector Concatenate1/1 -> SPI_Master_Transfer_To1/1
  Demux1/2 -> Data Type Conversion4/1
  Data Type Conversion4/1 -> Terminator1/1
  Demux1/1 -> Data Type Conversion3/1
  Chart/1(high) -> Data Type Conversion/1
  Chart/2(low) -> Data Type Conversion1/1
  Data Type Conversion/1 -> Vector Concatenate1/1
  Data Type Conversion1/1 -> Vector Concatenate1/2

== system ZT_VehCtrl_18B_CAN/Initialization & SPI timer1/CS2 CANB ==
  Action Port : ActionPort  ActionType=then
  Constant : Constant  Value=2
  Constant1 : Constant  Value=7
  Data Type Conversion : DataTypeConversion  OutDataTypeStr=uint8
  Data Type Conversion1 : DataTypeConversion  OutDataTypeStr=uint8
  Data Type Conversion2 : DataTypeConversion
  Data Type Conversion3 : DataTypeConversion
  Demux2 : Demux  Outputs=2
  SPI_Master_Transfer_To2 : mbd_mpc574x_ec_toolbox/Communication Blocks/SPI Blocks/SPI_Master_Transfer  Priority=2  InstanceNumber=3  xfermode=Non blocking  timeout=50  spi_upd=on  WhichPCS=2
  Terminator : Terminator
  Terminator1 : Terminator
  Vector Concatenate2 : Concatenate
  wires:
  Vector Concatenate2/1 -> SPI_Master_Transfer_To2/1
  Demux2/2 -> Data Type Conversion1/1
  Data Type Conversion2/1 -> Vector Concatenate2/2
  SPI_Master_Transfer_To2/1 -> Demux2/1
  Data Type Conversion1/1 -> Terminator1/1
  Data Type Conversion/1 -> Terminator/1
  Demux2/1 -> Data Type Conversion/1
  Data Type Conversion3/1 -> Vector Concatenate2/1
  Constant/1 -> Data Type Conversion3/1
  Constant1/1 -> Data Type Conversion2/1

== system ZT_VehCtrl_18B_CAN/Initialization & SPI timer1/CS3 LS ==
  note: 80-0101 0000 - 对A组端口控制模式进行设置
      | 96-0110 0000 - 对B组端口控制模式进行设置
      | 40-0010 1100 -使用SPI控制端口
      |
      | 其中端口1,2,5,6即为复用PWM端口，这里设置为引脚控制（A组），其余端口设置为SPI控制
  Action Port : ActionPort  ActionType=then
  Chart : Stateflow chart  TreatAsAtomicUnit=on
  Data Type Conversion : DataTypeConversion  OutDataTypeStr=uint8
  Data Type Conversion1 : DataTypeConversion  OutDataTypeStr=uint8
  Data Type Conversion2 : DataTypeConversion
  Data Type Conversion3 : DataTypeConversion
  Demux2 : Demux  Outputs=2
  Manual Switch : ManualSwitch  CurrentSetting=0
  PIN : Constant  Value=2
  SPI : Constant  Value=0
  SPI_Master_Transfer_To2 : mbd_mpc574x_ec_toolbox/Communication Blocks/SPI Blocks/SPI_Master_Transfer  Priority=2  InstanceNumber=3  xfermode=Non blocking  timeout=50  spi_upd=on  WhichPCS=3
  Subsystem : Subsystem  Commented=on
  Terminator2 : Terminator
  Terminator3 : Terminator
  Vector Concatenate1 : Concatenate
  wires:
  Data Type Conversion1/1 -> Terminator3/1
  Data Type Conversion/1 -> Terminator2/1
  Demux2/1 -> Data Type Conversion/1
  SPI_Master_Transfer_To2/1 -> Demux2/1
  Demux2/2 -> Data Type Conversion1/1
  Chart/2(low) -> Data Type Conversion3/1
  Vector Concatenate1/1 -> SPI_Master_Transfer_To2/1
  Data Type Conversion2/1 -> Vector Concatenate1/1
  Data Type Conversion3/1 -> Vector Concatenate1/2
  Chart/1(high) -> Data Type Conversion2/1
  PIN/1 -> Manual Switch/2
  SPI/1 -> Manual Switch/1
  Manual Switch/1 -> [Mode]
  [Mode] -> Chart/1(mode)

== system ZT_VehCtrl_18B_CAN/Initialization & SPI timer1/CS5 LS ==
  Action Port : ActionPort  ActionType=then
  Chart : Stateflow chart  TreatAsAtomicUnit=on
  Data Type Conversion{,1,3..4} (4 alike) : DataTypeConversion
  Demux1 : Demux  Outputs=2
  SPI_Master_Transfer_To1 : mbd_mpc574x_ec_toolbox/Communication Blocks/SPI Blocks/SPI_Master_Transfer  Priority=2  InstanceNumber=0  xfermode=Non blocking  timeout=50  spi_upd=on  WhichPCS=1
  Subsystem : Subsystem  Commented=on
  Terminator : Terminator
  Terminator1 : Terminator
  Vector Concatenate1 : Concatenate
  wires:
  SPI_Master_Transfer_To1/1 -> Demux1/1
  Demux1/1 -> Data Type Conversion3/1
  Data Type Conversion3/1 -> Terminator/1
  Demux1/2 -> Data Type Conversion4/1
  Data Type Conversion4/1 -> Terminator1/1
  Chart/2(low) -> Data Type Conversion1/1
  Vector Concatenate1/1 -> SPI_Master_Transfer_To1/1
  Data Type Conversion/1 -> Vector Concatenate1/1
  Data Type Conversion1/1 -> Vector Concatenate1/2
  Chart/1(high) -> Data Type Conversion/1

== system ZT_VehCtrl_18B_CAN/SPI_EEPROM/SPI_read ==
  Action Port : ActionPort
  "Address_High " : Constant  Value=hex2dec('FF')  OutDataTypeStr=uint8
  Address_Low : Constant  Value=hex2dec('FF')
  Bitwise AND : simulink/Logic and Bit Operations/Bitwise Operator  logicop=AND  UseBitMask=on  BitMask=hex2dec('00FF')  BitMaskRealWorld=Stored Integer
  Constant : Constant  Value=0
  Data Store Write : DataStoreWrite  DataStoreName=A_read
  Data Type Conversion{,1,3..8} (8 alike) : DataTypeConversion  OutDataTypeStr=uint8
  Data Type Conversion2 : DataTypeConversion
  Demux1 : Demux
  SPI_Master_Transfer_To1 : mbd_mpc574x_ec_toolbox/Communication Blocks/SPI Blocks/SPI_Master_Transfer  Priority=2  InstanceNumber=0  xfermode=Non blocking  timeout=50  spi_upd=on  WhichPCS=0
  Terminator : Terminator
  Terminator1 : Terminator
  Terminator2 : Terminator
  Vector Concatenate1 : Concatenate  NumInputs=4
  read_set : Constant  Value=3  OutDataTypeStr=uint8
  wires:
  "Address_High "/1 -> Data Type Conversion1/1
  read_set/1 -> Data Type Conversion/1
  Data Type Conversion1/1 -> Vector Concatenate1/2  "d1"
  Data Type Conversion/1 -> Vector Concatenate1/1  "d0"
  Address_Low/1 -> Data Type Conversion6/1
  Demux1/2 -> Data Type Conversion4/1
  Vector Concatenate1/1 -> SPI_Master_Transfer_To1/1
  Demux1/1 -> Data Type Conversion3/1
  SPI_Master_Transfer_To1/1 -> Demux1/1
  Data Type Conversion3/1 -> Terminator/1  "r0"
  Data Type Conversion8/1 -> Bitwise AND/1  "r3"
  Bitwise AND/1 -> Data Type Conversion2/1
  Data Type Conversion2/1 -> Data Store Write/1
  Constant/1 -> Data Type Conversion7/1
  Data Type Conversion6/1 -> Vector Concatenate1/3  "d2"
  Data Type Conversion7/1 -> Vector Concatenate1/4  "d3"
  Demux1/3 -> Data Type Conversion5/1
  Data Type Conversion4/1 -> Terminator1/1  "r1"
  Data Type Conversion5/1 -> Terminator2/1  "r2"
  Demux1/4 -> Data Type Conversion8/1

== system ZT_VehCtrl_18B_CAN/SPI_EEPROM/SPI_write ==
  Action Port : ActionPort
  Data Store Memory : DataStoreMemory  DataStoreName=Write_Ctrl  ReadBeforeWriteMsg=warning  WriteAfterWriteMsg=warning  WriteAfterReadMsg=warning  InitialValue=1  ShowAdditionalParam=off  OutDataTypeStr=uint8
      settings: RTWStateStorageClass=ExportedGlobal
  Data Store Read : DataStoreRead  DataStoreName=Write_Ctrl
  SPI_enable : Subsystem  TreatAsAtomicUnit=on
  SPI_write : Subsystem  TreatAsAtomicUnit=on
  Switch Case : SwitchCase  CaseConditions={1,2}  ShowDefaultCase=off
  wires:
  Data Store Read/1 -> Switch Case/1
  Switch Case/2 -> SPI_write/Action
  Switch Case/1 -> SPI_enable/Action

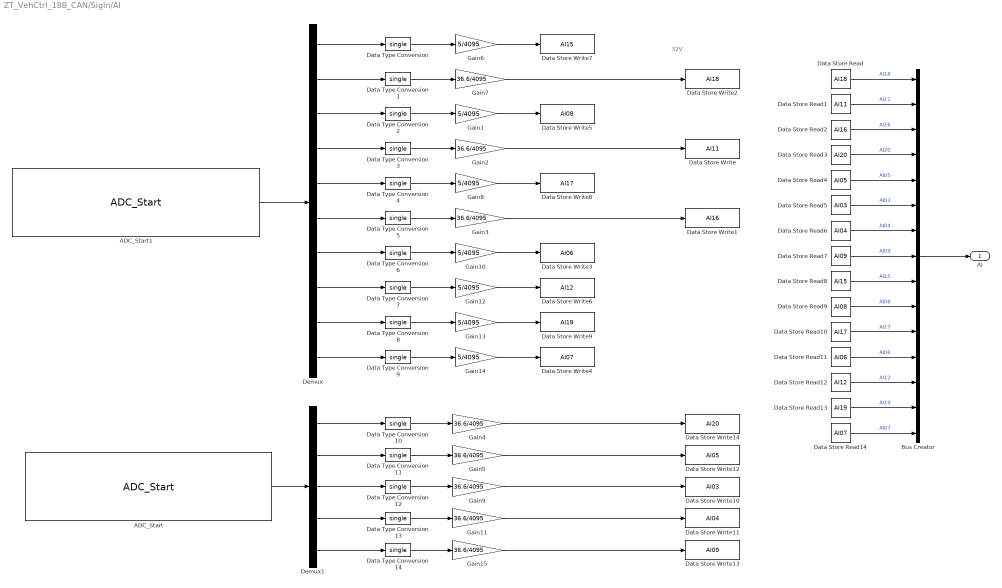
== system ZT_VehCtrl_18B_CAN/SigIn/AI ==
  note: 32V
  ADC_Start : mbd_mpc574x_ec_toolbox/Motor Control Blocks/ADC Blocks/ADC_Start  adc_instance=1  interrupt=off  presample=off
  ADC_Start1 : mbd_mpc574x_ec_toolbox/Motor Control Blocks/ADC Blocks/ADC_Start  adc_instance=0  interrupt=off  presample=off
  Bus Creator : BusCreator  Inputs=15
  Data Store Read : DataStoreRead  DataStoreName=AI18
  Data Store Read1 : DataStoreRead  DataStoreName=AI11
  Data Store Read10 : DataStoreRead  DataStoreName=AI17
  Data Store Read11 : DataStoreRead  DataStoreName=AI06
  Data Store Read12 : DataStoreRead  DataStoreName=AI12
  Data Store Read13 : DataStoreRead  DataStoreName=AI19
  Data Store Read14 : DataStoreRead  DataStoreName=AI07
  Data Store Read2 : DataStoreRead  DataStoreName=AI16
  Data Store Read3 : DataStoreRead  DataStoreName=AI20
  Data Store Read4 : DataStoreRead  DataStoreName=AI05
  Data Store Read5 : DataStoreRead  DataStoreName=AI03
  Data Store Read6 : DataStoreRead  DataStoreName=AI04
  Data Store Read7 : DataStoreRead  DataStoreName=AI09
  Data Store Read8 : DataStoreRead  DataStoreName=AI15
  Data Store Read9 : DataStoreRead  DataStoreName=AI08
  Data Store Write : DataStoreWrite  DataStoreName=AI11
  Data Store Write1 : DataStoreWrite  DataStoreName=AI16
  Data Store Write10 : DataStoreWrite  DataStoreName=AI03
  Data Store Write11 : DataStoreWrite  DataStoreName=AI04
  Data Store Write12 : DataStoreWrite  DataStoreName=AI05
  Data Store Write13 : DataStoreWrite  DataStoreName=AI09
  Data Store Write14 : DataStoreWrite  DataStoreName=AI20
  Data Store Write2 : DataStoreWrite  DataStoreName=AI18
  Data Store Write3 : DataStoreWrite  DataStoreName=AI06
  Data Store Write4 : DataStoreWrite  DataStoreName=AI07
  Data Store Write5 : DataStoreWrite  DataStoreName=AI08
  Data Store Write6 : DataStoreWrite  DataStoreName=AI12
  Data Store Write7 : DataStoreWrite  DataStoreName=AI15
  Data Store Write8 : DataStoreWrite  DataStoreName=AI17
  Data Store Write9 : DataStoreWrite  DataStoreName=AI19
  Data Type Conversion{,1..14} (15 alike) : DataTypeConversion  OutDataTypeStr=single
  Demux : Demux  Outputs=10
  Demux1 : Demux  Outputs=5
  Gain{1,6,8,10,12..14} (7 alike) : Gain  Gain=5/4095
  Gain{2..5,7,9,11,15} (8 alike) : Gain  Gain=36.6/4095  OutDataTypeStr=single
  AI : Outport
  wires:
  Demux/4 -> Data Type Conversion3/1
  ADC_Start1/1 -> Demux/1
  Demux/7 -> Data Type Conversion6/1
  Demux1/4 -> Data Type Conversion13/1
  Demux1/3 -> Data Type Conversion12/1
  ADC_Start/1 -> Demux1/1
  Demux1/2 -> Data Type Conversion11/1
  Demux1/5 -> Data Type Conversion14/1
  Demux1/1 -> Data Type Conversion10/1
  Demux/1 -> Data Type Conversion/1
  Demux/3 -> Data Type Conversion2/1
  Demux/2 -> Data Type Conversion1/1
  Demux/5 -> Data Type Conversion4/1
  Demux/8 -> Data Type Conversion7/1
  Demux/9 -> Data Type Conversion8/1
  Demux/10 -> Data Type Conversion9/1
  Demux/6 -> Data Type Conversion5/1
  Data Type Conversion/1 -> Gain6/1
  Gain6/1 -> Data Store Write7/1
  Data Type Conversion1/1 -> Gain7/1
  Data Type Conversion2/1 -> Gain1/1
  Data Type Conversion3/1 -> Gain2/1
  Data Type Conversion4/1 -> Gain8/1
  Data Type Conversion5/1 -> Gain3/1
  Data Type Conversion6/1 -> Gain10/1
  Data Type Conversion7/1 -> Gain12/1
  Data Type Conversion8/1 -> Gain13/1
  Data Type Conversion9/1 -> Gain14/1
  Data Type Conversion10/1 -> Gain4/1
  Data Type Conversion11/1 -> Gain5/1
  Data Type Conversion12/1 -> Gain9/1
  Data Type Conversion13/1 -> Gain11/1
  Data Type Conversion14/1 -> Gain15/1
  Gain7/1 -> Data Store Write2/1
  Gain1/1 -> Data Store Write5/1
  Gain2/1 -> Data Store Write/1
  Gain8/1 -> Data Store Write8/1
  Gain3/1 -> Data Store Write1/1
  Gain10/1 -> Data Store Write3/1
  Gain12/1 -> Data Store Write6/1
  Gain13/1 -> Data Store Write9/1
  Gain14/1 -> Data Store Write4/1
  Gain4/1 -> Data Store Write14/1
  Gain5/1 -> Data Store Write12/1
  Gain9/1 -> Data Store Write10/1
  Gain11/1 -> Data Store Write11/1
  Gain15/1 -> Data Store Write13/1
  Data Store Read/1 -> Bus Creator/1  "AI18"
  Data Store Read1/1 -> Bus Creator/2  "AI11"
  Data Store Read2/1 -> Bus Creator/3  "AI16"
  Data Store Read3/1 -> Bus Creator/4  "AI20"
  Data Store Read4/1 -> Bus Creator/5  "AI05"
  Data Store Read5/1 -> Bus Creator/6  "AI03"
  Data Store Read6/1 -> Bus Creator/7  "AI04"
  Data Store Read7/1 -> Bus Creator/8  "AI09"
  Data Store Read8/1 -> Bus Creator/9  "AI15"
  Data Store Read9/1 -> Bus Creator/10  "AI08"
  Data Store Read10/1 -> Bus Creator/11  "AI17"
  Data Store Read11/1 -> Bus Creator/12  "AI06"
  Data Store Read12/1 -> Bus Creator/13  "AI12"
  Data Store Read13/1 -> Bus Creator/14  "AI19"
  Data Store Read14/1 -> Bus Creator/15  "AI07"
  Bus Creator/1 -> AI/1
